simulink model "ecu_diag"  (R2026a)
settings: Solver=FixedStepDiscrete  StopTime=10  FixedStep=0.001  SampleTimeConstraint=STIndependent
Description:
  | Engine-side diagnoses and coolant protection, 14 conditions. Source of truth for firmware/gen/ecu_diag.
settings Model: Creator=jj1001000  LastModifiedBy=jj1001000
settings OptimizationCC: DefaultUnderspecifiedDataType=single
settings DebuggingCC: ParameterPrecisionLossMsg=none
settings HardwareCC: ProdLargestAtomicInteger=Long  ProdLargestAtomicFloat=Double  ProdHWDeviceType=ARM Compatible->ARM Cortex-M
settings RTWCC: SystemTargetFile=ert.tlc  GenCodeOnly=on  Description=Embedded Coder
settings ERTTargetCC: UtilityFuncGeneration=Shared location  IncludeMdlTerminateFcn=off  CodeInterfacePackaging=Reusable function  SupportNonFinite=off

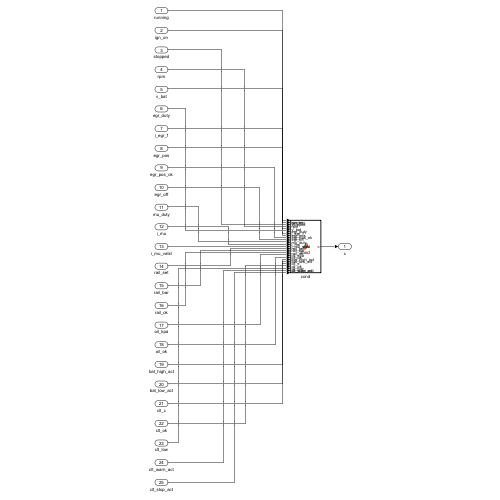
[thumbnail: Simulink's stored preview of the top-level diagram]
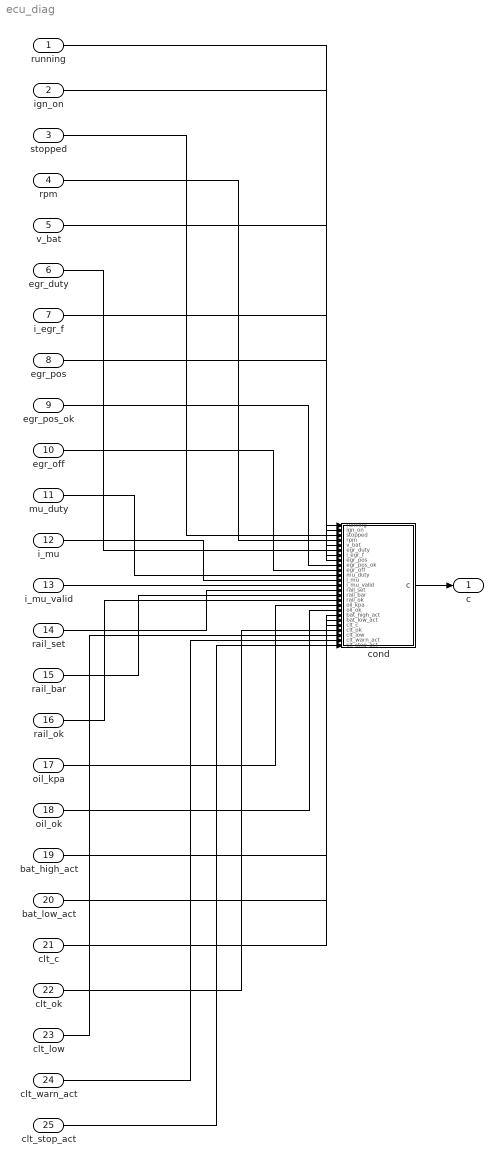
== system ecu_diag ==
  running : Inport  OutDataTypeStr=uint8
  ign_on : Inport  Port=2  OutDataTypeStr=uint8
  stopped : Inport  Port=3  OutDataTypeStr=uint8
  rpm : Inport  Port=4  OutDataTypeStr=single
  v_bat : Inport  Port=5  OutDataTypeStr=single
  egr_duty : Inport  Port=6  OutDataTypeStr=single
  i_egr_f : Inport  Port=7  OutDataTypeStr=single
  egr_pos : Inport  Port=8  OutDataTypeStr=single
  egr_pos_ok : Inport  Port=9  OutDataTypeStr=uint8
  egr_off : Inport  Port=10  OutDataTypeStr=uint8
  mu_duty : Inport  Port=11  OutDataTypeStr=single
  i_mu : Inport  Port=12  OutDataTypeStr=single
  i_mu_valid : Inport  Port=13  OutDataTypeStr=uint8
  rail_set : Inport  Port=14  OutDataTypeStr=single
  rail_bar : Inport  Port=15  OutDataTypeStr=single
  rail_ok : Inport  Port=16  OutDataTypeStr=uint8
  oil_kpa : Inport  Port=17  OutDataTypeStr=single
  oil_ok : Inport  Port=18  OutDataTypeStr=uint8
  bat_high_act : Inport  Port=19  OutDataTypeStr=uint8
  bat_low_act : Inport  Port=20  OutDataTypeStr=uint8
  clt_c : Inport  Port=21  OutDataTypeStr=single
  clt_ok : Inport  Port=22  OutDataTypeStr=uint8
  clt_low : Inport  Port=23  OutDataTypeStr=uint8
  clt_warn_act : Inport  Port=24  OutDataTypeStr=uint8
  clt_stop_act : Inport  Port=25  OutDataTypeStr=uint8
  cond : MATLAB Function  TreatAsAtomicUnit=on
  c : Outport  OutDataTypeStr=uint8
  wires:
  running/1 -> cond/1(running)
  ign_on/1 -> cond/2(ign_on)
  stopped/1 -> cond/3(stopped)
  rpm/1 -> cond/4(rpm)
  v_bat/1 -> cond/5(v_bat)
  egr_pos_ok/1 -> cond/9(egr_pos_ok)
  egr_duty/1 -> cond/6(egr_duty)
  i_egr_f/1 -> cond/7(i_egr_f)
  egr_pos/1 -> cond/8(egr_pos)
  i_mu_valid/1 -> cond/13(i_mu_valid)
  i_mu/1 -> cond/12(i_mu)
  mu_duty/1 -> cond/11(mu_duty)
  egr_off/1 -> cond/10(egr_off)
  oil_kpa/1 -> cond/17(oil_kpa)
  rail_ok/1 -> cond/16(rail_ok)
  rail_bar/1 -> cond/15(rail_bar)
  rail_set/1 -> cond/14(rail_set)
  clt_c/1 -> cond/21(clt_c)
  bat_low_act/1 -> cond/20(bat_low_act)
  bat_high_act/1 -> cond/19(bat_high_act)
  oil_ok/1 -> cond/18(oil_ok)
  clt_stop_act/1 -> cond/25(clt_stop_act)
  clt_warn_act/1 -> cond/24(clt_warn_act)
  clt_low/1 -> cond/23(clt_low)
  clt_ok/1 -> cond/22(clt_ok)
  cond/1(c) -> c/1

== matlab function ecu_diag/cond ==
  data: running input uint8; c output uint8; ign_on input uint8; stopped input uint8; rpm input single; v_bat input single; egr_duty input single; i_egr_f input single; egr_pos input single; egr_pos_ok input uint8; egr_off input uint8; mu_duty input single; i_mu input single; i_mu_valid input uint8; rail_set input single; rail_bar input single; rail_ok input uint8; oil_kpa input single; oil_ok input uint8; bat_high_act input uint8; bat_low_act input uint8; clt_c input single; clt_ok input uint8; clt_low input uint8; clt_warn_act input uint8; clt_stop_act input uint8
function c = cond(running, ign_on, stopped, rpm, v_bat, egr_duty, i_egr_f, egr_pos, egr_pos_ok, egr_off, mu_duty, i_mu, i_mu_valid, rail_set, rail_bar, rail_ok, oil_kpa, oil_ok, bat_high_act, bat_low_act, clt_c, clt_ok, clt_low, clt_warn_act, clt_stop_act)
%#codegen
c = zeros(14, 1, 'uint8');
bat_known = v_bat >= single(1);
% EGR: running, the stall guard not holding it off, a workable battery
% (unknown counts as fine: production may not measure it)
egr = running ~= 0 && egr_off == 0 && ...
      (~bat_known || (v_bat >= single(10) && v_bat <= single(15)));
d = abs(egr_duty);
c(1) = uint8(egr && d > single(0.200000003) && i_egr_f <= single(0.100000001));
c(2) = uint8(egr && egr_pos_ok ~= 0 && d < single(0.0500000007) && egr_pos > single(35));
c(3) = uint8(egr && egr_pos_ok ~= 0 && egr_duty >= single(0.899999976) && egr_pos < single(35));
% the metering valve: only where its current is measured
c(4) = uint8(i_mu_valid ~= 0 && mu_duty * v_bat / single(6.90999985) > single(0.25) && i_mu < single(0.0500000007));
c(5) = uint8(i_mu_valid ~= 0 && i_mu > single(3));
dev = abs(rail_set - rail_bar);
c(6) = uint8(running ~= 0 && rail_ok ~= 0 && dev > single(150) && dev > single(0.25) * rail_set);
c(7) = uint8(running ~= 0 && rpm > single(1590));
% stopped, yet oil pressure says turning / is implausible
c(8) = uint8(ign_on ~= 0 && stopped ~= 0 && oil_ok ~= 0 && oil_kpa > single(200));
c(9) = uint8(ign_on ~= 0 && stopped ~= 0 && oil_ok ~= 0 && oil_kpa > single(100) && oil_kpa <= single(200));
if bat_high_act ~= 0
    bh = single(14.5);
else
    bh = single(15);
end
c(10) = uint8(ign_on ~= 0 && bat_known && v_bat > bh);
% running only: cranking pulls any battery below 10 V
if bat_low_act ~= 0
    bl = single(10);
else
    bl = single(9.5);
end
c(11) = uint8(running ~= 0 && bat_known && v_bat < bl);
% coolant: only from a good sensor (a faulted one reads its default)
if clt_warn_act ~= 0
    cw = single(98);
else
    cw = single(100);
end
c(12) = uint8(ign_on ~= 0 && clt_ok ~= 0 && clt_c > cw);
if clt_stop_act ~= 0
    cs = single(102);
else
    cs = single(104);
end
c(13) = uint8(ign_on ~= 0 && clt_ok ~= 0 && clt_c > cs);
c(14) = uint8(ign_on ~= 0 && clt_low ~= 0);
